simulink model "AFC1_FFNN_trainrp_15_15_15_15_ep_1000_Nor_20250519"  (R2021a)
settings: Solver=ode15s  StartTime=0.0  StopTime=T  MaxStep=.01  RelTol=1e-3
undefined symbols (not defined in the file or in its folder): AF_sensor_tol, fault_time, fuel_inj_tol, kappa_tol, MAF_sensor_tol, pump_tol, tau_ww_tol, x_gain, x_offset, y_gain, y_offset
libraries: neural x66
(part 1 of 3)
Description:
  | Modeling Engine Timing Using Triggered Subsystems
  | 
  | This example presents a model of a four-cylinder spark ignition engine
  | and demonstrates Simulink(R) capabilities to model an internal combustion
  | engine from the throttle to the crankshaft output. We used well-defined
  | physical principles supplemented, where appropriate, with empirical
  | relationships that describe the systems dynamic behavior without
  | introducing unnecessary complexity.
settings Model: ExtModeTrigMode=oneshot  ExtModeArmWhenConnect=off  ExtModeAutoUpdateStatusClock=off  Creator=The MathWorks Inc.  LastModifiedBy=deyun
settings SolverCC: ZeroCrossControl=DisableAll  AlgebraicLoopSolver=TrustRegion
settings DataIOCC: ExternalInput=[t__, u__]  LoadExternalInput=on  SaveFormat=StructureWithTime  SignalLogging=off  DSMLogging=off  ReturnWorkspaceOutputs=off
settings OptimizationCC: BlockReduction=off  BooleanDataType=off  LifeSpan=inf
settings DebuggingCC: SaveWithParameterizedLinksMsg=none  UnderspecifiedInitializationDetection=Classic  MergeDetectMultiDrivingBlocksExec=none  SignalResolutionControl=TryResolveAllWithWarning  ParameterPrecisionLossMsg=none  SFUnexpectedBacktrackingDiag=warning  SFNoUnconditionalDefaultTransitionDiag=warning  SFExecutionAtInitializationDiag=none  ArithmeticOperatorsInVariantConditions=warning
settings HardwareCC: ProdBitPerPointer=32  ProdBitPerSizeT=32  ProdBitPerPtrDiffT=32  ProdLargestAtomicFloat=None  ProdIntDivRoundTo=Undefined  ProdEndianess=Unspecified  ProdWordSize=32  ProdHWDeviceType=32-bit Generic  TargetBitPerLong=64  TargetBitPerPointer=64  TargetBitPerSizeT=64  TargetBitPerPtrDiffT=64  TargetLongLongMode=on  TargetIntDivRoundTo=Zero  TargetEndianess=LittleEndian  TargetWordSize=64  TargetHWDeviceType=MATLAB Host  ProdEqTarget=off
settings ModelReferenceCC: PropagateSignalLabelsOutOfModel=off
settings SFSimCC: SimUseLocalCustomCode=off  CustomCodeUndefinedFunction=UseInterfaceOnly
settings RTWCC: RTWUseLocalCustomCode=off
settings CodeAppCC: StateflowObjectComments=on
settings GRTTargetCC: TargetLangStandard=C89/C90 (ANSI)
settings ConfigComp: CovMetricSettings=d  CovSaveCumulativeToWorkspaceVar=on  CovSaveSingleToWorkspaceVar=on  CovExternalEMLEnable=off

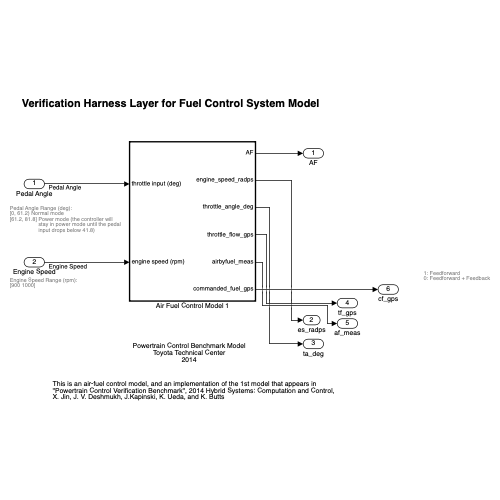
[thumbnail: Simulink's stored preview of the top-level diagram]
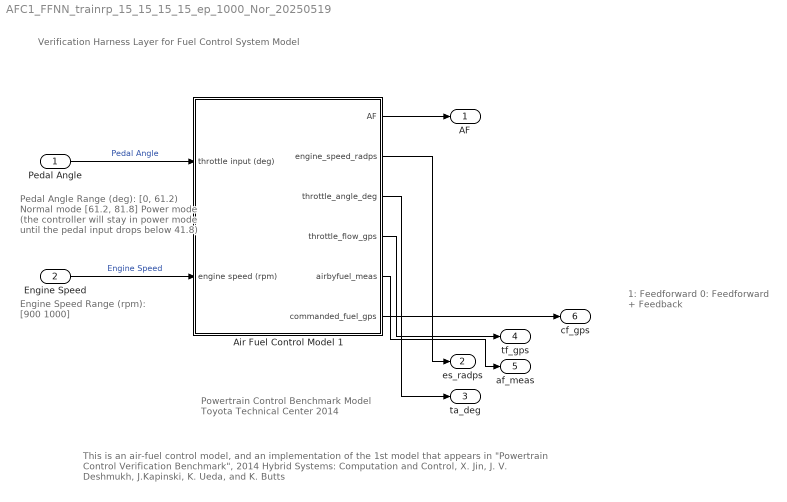
== system AFC1_FFNN_trainrp_15_15_15_15_ep_1000_Nor_20250519 ==
  note: 1: Feedforward
      | 0: Feedforward + Feedback
  note: Pedal Angle Range (deg):
      | [0, 61.2) Normal mode
      | [61.2, 81.8] Power mode (the controller will
      |                    stay in power mode until the pedal
      |                    input drops below 41.8)
  note: This is an air-fuel control model, and an implementation of the 1st model that appears in
      | "Powertrain Control Verification Benchmark", 2014 Hybrid Systems: Computation and Control,
      | X. Jin, J. V. Deshmukh, J.Kapinski, K. Ueda, and K. Butts
  note: Engine Speed Range (rpm):
      | [900 1000]
  note: Powertrain Control Benchmark Model
      | Toyota Technical Center
      | 2014
  note: Verification Harness Layer for Fuel Control System Model
  Pedal Angle : Inport  Interpolate=off
  Engine Speed : Inport  Port=2  Interpolate=off
  Air Fuel Control Model 1 : Subsystem  Priority=1  TreatAsAtomicUnit=on
  AF : Outport  VectorParamsAs1DForOutWhenUnconnected=off
  es_radps : Outport  Port=2
  ta_deg : Outport  Port=3
  tf_gps : Outport  Port=4
  af_meas : Outport  Port=5
  cf_gps : Outport  Port=6
  wires:
  Air Fuel Control Model 1/1(AF) -> AF/1
  Pedal Angle/1 -> Air Fuel Control Model 1/1(throttle input (deg))  "Pedal Angle"
  Engine Speed/1 -> Air Fuel Control Model 1/2(engine speed (rpm))  "Engine Speed"
  Air Fuel Control Model 1/2(engine_speed_radps) -> es_radps/1
  Air Fuel Control Model 1/3(throttle_angle_deg) -> ta_deg/1
  Air Fuel Control Model 1/4(throttle_flow_gps) -> tf_gps/1
  Air Fuel Control Model 1/5(airbyfuel_meas) -> af_meas/1
  Air Fuel Control Model 1/6(commanded_fuel_gps) -> cf_gps/1

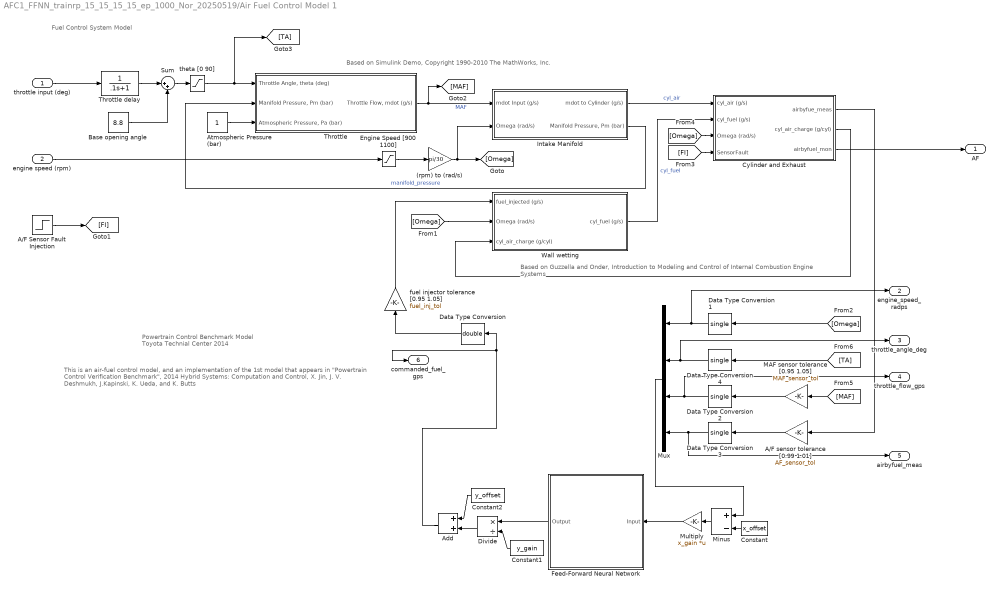
== system AFC1_FFNN_trainrp_15_15_15_15_ep_1000_Nor_20250519/Air Fuel Control Model 1 ==
  note: Based on Simulink Demo, Copyright 1990-2010 The MathWorks, Inc.
  note: Based on Guzzella and Onder, Introduction to Modeling and Control of Internal Combustion Engine Systems
  note: Fuel Control System Model
  note: This is an air-fuel control model, and an implementation of the 1st model that appears in
      | "Powertrain Control Verification Benchmark", 2014 Hybrid Systems: Computation and Control,
      | X. Jin, J. V. Deshmukh, J.Kapinski, K. Ueda, and K. Butts
  note: Powertrain Control Benchmark Model
      | Toyota Technial Center
      | 2014
  throttle input (deg) : Inport  Description=[0, 81.2]
      settings: AttributesFormatString=%<Description>
  engine speed (rpm) : Inport  Description=[900,1100]  Port=2
      settings: AttributesFormatString=%<Description>
  (rpm) to (rad/s) : Gain  Gain=pi/30
  A/F Sensor Fault Injection : Step  Time=fault_time  SampleTime=0
      settings: AttributesFormatString=1: Failure\n0: Normal
  A/F sensor tolerance [0.99 1.01] : Gain  Gain=AF_sensor_tol
  Add : Sum
  Atmospheric Pressure (bar) : Constant
  Base opening angle : Constant  Value=8.8
  Constant : Constant  Value=x_offset
  Constant1 : Constant  Value=y_gain
  Constant2 : Constant  Value=y_offset
  Cylinder and Exhaust : Subsystem
  Data Type Conversion : DataTypeConversion  OutDataTypeStr=double
  Data Type Conversion{1..4} (4 alike) : DataTypeConversion  OutDataTypeStr=single
  Divide : Product  Inputs=*/
  Engine Speed [900 1100] : Saturate  UpperLimit=1100  LowerLimit=900
  Feed-Forward Neural Network : Subsystem
      mask help: Feed-Forward Neural Network
      mask Display: e = 0.06;c1 = [120 150 230]/255;c2 = ([120 150 230]+0)/383;c3 = ([120 150 230]+128)/383;patch([0 1 1 0],[0 0 1 1],c1);patch([0 1 1 1-e 1-e 0+e],[0 0 1 1-e 0+e 0+e],c2);patch([0 0 1 1-e 0+e 0+e],[0 1 1 1-e 1-e 0+e],c3);plot([0 1 1 0 0],[0 0 1 1 0]);fprintf('NNET');port_label('input',1,' Input');port_label('output',1,'Output ');
  Intake Manifold : Subsystem
  MAF sensor tolerance [0.95 1.05] : Gain  Gain=MAF_sensor_tol
  Minus : Sum  Inputs=+-
  Multiply : Gain  Gain=x_gain  Multiplication=Matrix(K*u)
  Mux : Mux
  Sum : Sum  Inputs=|++
  Throttle : Subsystem
  Throttle delay : TransferFcn  Denominator=[.1 1]
  Wall wetting : Subsystem
  fuel injector tolerance [0.95 1.05] : Gain  Gain=fuel_inj_tol
  theta [0 90] : Saturate  UpperLimit=90  LowerLimit=0
  AF : Outport  VectorParamsAs1DForOutWhenUnconnected=off
  engine_speed_radps : Outport  Port=2
  throttle_angle_deg : Outport  Port=3
  throttle_flow_gps : Outport  Port=4
  airbyfuel_meas : Outport  Port=5
  commanded_fuel_gps : Outport  Port=6
  wires:
  (rpm) to (rad/s)/1 -> [Omega], Intake Manifold/2(Omega (rad/s))
  Data Type Conversion/1 -> fuel injector tolerance [0.95 1.05]/1
  theta [0 90]/1 -> Throttle/1("Throttle Angle, theta (deg)"), [TA]
  Engine Speed [900 1100]/1 -> (rpm) to (rad/s)/1
  Cylinder and Exhaust/3("airbyfuel_mon ") -> AF/1
  A/F sensor tolerance [0.99 1.01]/1 -> Data Type Conversion3/1
  [MAF] -> MAF sensor tolerance [0.95 1.05]/1
  Cylinder and Exhaust/1(airbyfue_meas) -> A/F sensor tolerance [0.99 1.01]/1
  Throttle/1("Throttle Flow, mdot (g/s)") -> [MAF], Intake Manifold/1(mdot Input (g/s))  "MAF"
  Intake Manifold/2("Manifold Pressure, Pm (bar)") -> Throttle/2("Manifold Pressure, Pm (bar)")  "manifold_pressure"
  Atmospheric Pressure (bar)/1 -> Throttle/3("Atmospheric Pressure, Pa (bar) ")
  Wall wetting/1(cyl_fuel (g/s)) -> Cylinder and Exhaust/2(cyl_fuel (g/s))  "cyl_fuel"
  Intake Manifold/1(mdot to Cylinder (g/s)) -> Cylinder and Exhaust/1(cyl_air (g/s))  "cyl_air"
  [Omega] -> Cylinder and Exhaust/3(Omega (rad/s))
  [Omega] -> Wall wetting/2(Omega (rad/s))
  Cylinder and Exhaust/2(cyl_air_charge (g/cyl)) -> Wall wetting/3(cyl_air_charge (g/cyl))
  [Omega] -> Data Type Conversion1/1
  fuel injector tolerance [0.95 1.05]/1 -> Wall wetting/1(fuel_injected (g/s))
  MAF sensor tolerance [0.95 1.05]/1 -> Data Type Conversion2/1
  Add/1 -> Data Type Conversion/1, commanded_fuel_gps/1
  A/F Sensor Fault Injection/1 -> [FI]
  [FI] -> Cylinder and Exhaust/4(SensorFault)
  [TA] -> Data Type Conversion4/1
  throttle input (deg)/1 -> Throttle delay/1
  engine speed (rpm)/1 -> Engine Speed [900 1100]/1
  Throttle delay/1 -> Sum/1
  Base opening angle/1 -> Sum/2
  Sum/1 -> theta [0 90]/1
  Data Type Conversion3/1 -> airbyfuel_meas/1, Mux/4
  Data Type Conversion4/1 -> Mux/2, throttle_angle_deg/1
  Data Type Conversion2/1 -> Mux/3, throttle_flow_gps/1
  Data Type Conversion1/1 -> Mux/1, engine_speed_radps/1
  Multiply/1 -> Feed-Forward Neural Network/1(Input)
  Constant/1 -> Minus/2
  Mux/1 -> Minus/1
  Minus/1 -> Multiply/1
  Constant2/1 -> Add/1
  Feed-Forward Neural Network/1(Output) -> Divide/1
  Constant1/1 -> Divide/2
  Divide/1 -> Add/2

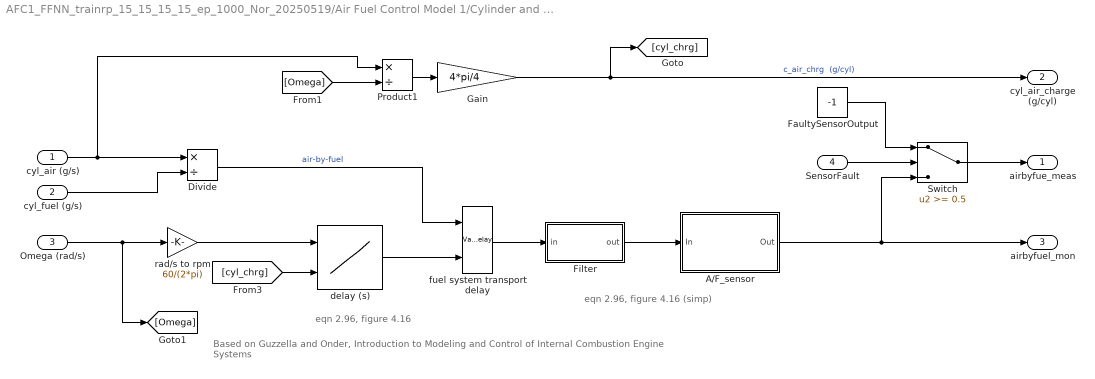
== system AFC1_FFNN_trainrp_15_15_15_15_ep_1000_Nor_20250519/Air Fuel Control Model 1/Cylinder and Exhaust ==
  note: Based on Guzzella and Onder, Introduction to Modeling and Control of Internal Combustion Engine Systems
  note: eqn 2.96, figure 4.16
  note: eqn 2.96, figure 4.16 (simp)
  cyl_air (g/s) : Inport
  cyl_fuel (g/s) : Inport  Port=2
  Omega (rad/s) : Inport  Port=3
  SensorFault : Inport  Port=4
  A/F_sensor : Subsystem
  Divide : Product  Inputs=*/
  FaultySensorOutput : Constant  Value=-1
  Filter : Subsystem
  Gain : Gain  Gain=4*pi/4
  Product1 : Product  Inputs=*/  RndMeth=Zero
  Switch : Switch  Threshold=0.5
  delay (s) : Lookup_n-D  BreakpointsForDimension1=[800,1000,1500,2000,3000]  BreakpointsForDimension2=[0.05,0.15,0.2,0.25]  Table=reshape([0.8,0.6,0.4,0.3,0.2,0.4,0.3,0.2,0.2,0.2,0.3,0.25,0.2,0.2,0.2,0.25,0.2,0.2,0.2,0.2],5,4)  UseLastTableValue=on  RndMeth=Simplest  InputSameDT=on
      settings: InputPortMap=u0,u1
  fuel system transport delay : VariableTransportDelay  VariableDelayType=Variable transport delay  MaximumDelay=10  InitialOutput=14.7  MaximumPoints=20480
  rad/s to rpm : Gain  Gain=60/(2*pi)
  airbyfue_meas : Outport  VectorParamsAs1DForOutWhenUnconnected=off
  cyl_air_charge (g/cyl) : Outport  Port=2  VectorParamsAs1DForOutWhenUnconnected=off
  "airbyfuel_mon " : Outport  Port=3  VectorParamsAs1DForOutWhenUnconnected=off
  wires:
  cyl_air (g/s)/1 -> Divide/1, Product1/1
  [Omega] -> Product1/2
  Product1/1 -> Gain/1
  Gain/1 -> [cyl_chrg], cyl_air_charge (g/cyl)/1  "c_air_chrg  (g/cyl)"
  [cyl_chrg] -> delay (s)/2
  cyl_fuel (g/s)/1 -> Divide/2
  Omega (rad/s)/1 -> [Omega], rad/s to rpm/1
  rad/s to rpm/1 -> delay (s)/1
  delay (s)/1 -> fuel system transport delay/2
  fuel system transport delay/1 -> Filter/1(in)
  Switch/1 -> airbyfue_meas/1
  Divide/1 -> fuel system transport delay/1  "air-by-fuel"
  Filter/1(out) -> A/F_sensor/1(In)
  FaultySensorOutput/1 -> Switch/1
  SensorFault/1 -> Switch/2
  A/F_sensor/1(Out) -> Switch/3, "airbyfuel_mon "/1

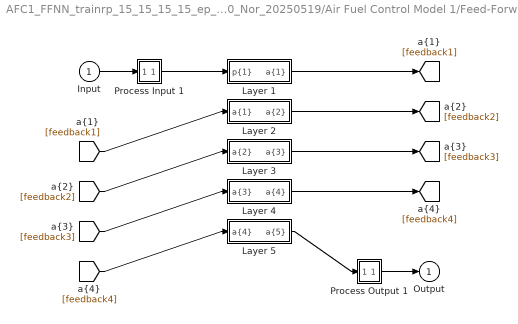
== system AFC1_FFNN_trainrp_15_15_15_15_ep_1000_Nor_20250519/Air Fuel Control Model 1/Feed-Forward Neural Network ==
  Input : Inport  PortDimensions=4
      mask Display: e = 0.06;c1 = [120 230 180]/255;c2 = ([120 230 180]+0)/(256+128);c3 = ([120 230 180]+128)/(256+128);patch([0 1 1 0],[0 0 1 1],c1);patch([0 1 1 1-e 1-e 0+e],[0 0 1 1-e 0+e 0+e],c2);patch([0 0 1 1-e 0+e 0+e],[0 1 1 1-e 1-e 0+e],c3);plot([0 1 1 0 0],[0 0 1 1 0]);
  Layer 1 : Subsystem
      mask Display: e = 0.06;c1 = [120 150 230]/255;c2 = ([120 150 230]+0)/383;c3 = ([120 150 230]+128)/383;patch([0 1 1 0],[0 0 1 1],c1);patch([0 1 1 1-e 1-e 0+e],[0 0 1 1-e 0+e 0+e],c2);patch([0 0 1 1-e 0+e 0+e],[0 1 1 1-e 1-e 0+e],c3);plot([0 1 1 0 0],[0 0 1 1 0]);
  Layer 2 : Subsystem
      mask Display: e = 0.06;c1 = [120 150 230]/255;c2 = ([120 150 230]+0)/383;c3 = ([120 150 230]+128)/383;patch([0 1 1 0],[0 0 1 1],c1);patch([0 1 1 1-e 1-e 0+e],[0 0 1 1-e 0+e 0+e],c2);patch([0 0 1 1-e 0+e 0+e],[0 1 1 1-e 1-e 0+e],c3);plot([0 1 1 0 0],[0 0 1 1 0]);
  Layer 3 : Subsystem
      mask Display: e = 0.06;c1 = [120 150 230]/255;c2 = ([120 150 230]+0)/383;c3 = ([120 150 230]+128)/383;patch([0 1 1 0],[0 0 1 1],c1);patch([0 1 1 1-e 1-e 0+e],[0 0 1 1-e 0+e 0+e],c2);patch([0 0 1 1-e 0+e 0+e],[0 1 1 1-e 1-e 0+e],c3);plot([0 1 1 0 0],[0 0 1 1 0]);
  Layer 4 : Subsystem
      mask Display: e = 0.06;c1 = [120 150 230]/255;c2 = ([120 150 230]+0)/383;c3 = ([120 150 230]+128)/383;patch([0 1 1 0],[0 0 1 1],c1);patch([0 1 1 1-e 1-e 0+e],[0 0 1 1-e 0+e 0+e],c2);patch([0 0 1 1-e 0+e 0+e],[0 1 1 1-e 1-e 0+e],c3);plot([0 1 1 0 0],[0 0 1 1 0]);
  Layer 5 : Subsystem
      mask Display: e = 0.06;c1 = [120 150 230]/255;c2 = ([120 150 230]+0)/383;c3 = ([120 150 230]+128)/383;patch([0 1 1 0],[0 0 1 1],c1);patch([0 1 1 1-e 1-e 0+e],[0 0 1 1-e 0+e 0+e],c2);patch([0 0 1 1-e 0+e 0+e],[0 1 1 1-e 1-e 0+e],c3);plot([0 1 1 0 0],[0 0 1 1 0]);
  Process Input 1 : Subsystem
      mask Display: e = 0.06;c1 = [120 150 230]/255;c2 = ([120 150 230]+0)/383;c3 = ([120 150 230]+128)/383;patch([0 1 1 0],[0 0 1 1],c1);patch([0 1 1 1-e 1-e 0+e],[0 0 1 1-e 0+e 0+e],c2);patch([0 0 1 1-e 0+e 0+e],[0 1 1 1-e 1-e 0+e],c3);plot([0 1 1 0 0],[0 0 1 1 0]);
  Process Output 1 : Subsystem
      mask Display: e = 0.06;c1 = [120 150 230]/255;c2 = ([120 150 230]+0)/383;c3 = ([120 150 230]+128)/383;patch([0 1 1 0],[0 0 1 1],c1);patch([0 1 1 1-e 1-e 0+e],[0 0 1 1-e 0+e 0+e],c2);patch([0 0 1 1-e 0+e 0+e],[0 1 1 1-e 1-e 0+e],c3);plot([0 1 1 0 0],[0 0 1 1 0]);
  Output : Outport  InitialOutput=0
      mask Display: e = 0.06;c1 = [120 230 180]/255;c2 = ([120 230 180]+0)/(256+128);c3 = ([120 230 180]+128)/(256+128);patch([0 1 1 0],[0 0 1 1],c1);patch([0 1 1 1-e 1-e 0+e],[0 0 1 1-e 0+e 0+e],c2);patch([0 0 1 1-e 0+e 0+e],[0 1 1 1-e 1-e 0+e],c3);plot([0 1 1 0 0],[0 0 1 1 0]);
  wires:
  Layer 5/1("a{5}") -> Process Output 1/1(a)
  [feedback4] -> Layer 5/1("a{4} ")
  Layer 4/1("a{4}") -> [feedback4]
  [feedback3] -> Layer 4/1("a{3} ")
  Layer 3/1("a{3}") -> [feedback3]
  [feedback2] -> Layer 3/1("a{2} ")
  Layer 2/1("a{2}") -> [feedback2]
  [feedback1] -> Layer 2/1("a{1} ")
  Layer 1/1("a{1}") -> [feedback1]
  Process Input 1/1(p) -> Layer 1/1("p{1}")
  Process Output 1/1(y) -> Output/1
  Input/1 -> Process Input 1/1(x)

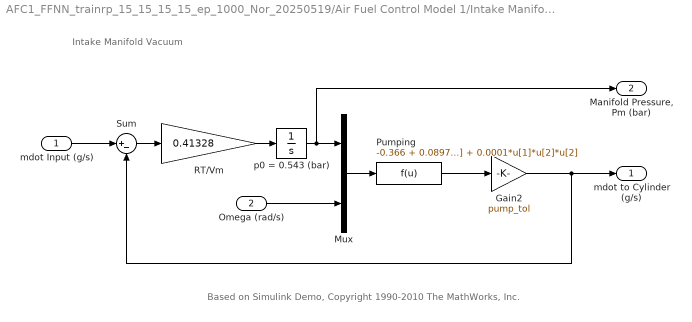
== system AFC1_FFNN_trainrp_15_15_15_15_ep_1000_Nor_20250519/Air Fuel Control Model 1/Intake Manifold ==
  note: Intake Manifold Vacuum
  note: Based on Simulink Demo, Copyright 1990-2010 The MathWorks, Inc.
  mdot Input (g/s) : Inport
  Omega (rad/s) : Inport  Port=2
  Gain2 : Gain  Gain=pump_tol  ParamDataTypeStr=single  OutDataTypeStr=Inherit: Inherit via back propagation  RndMeth=Simplest  SaturateOnIntegerOverflow=on
      settings: AttributesFormatString=pumping tolerance [0.9 1.1]
  Mux : Mux  Inputs=2
  Pumping : Fcn  Expr=-0.366 + 0.08979*u[1]*u[2] - 0.0337*u[2]*u[1]*u[1] + 0.0001*u[1]*u[2]*u[2]
  RT/Vm : Gain  Gain=0.41328  SaturateOnIntegerOverflow=on  OutDataTypeStr=Inherit: Same as input  ParamDataTypeStr=Inherit: Same as input
  Sum : Sum  Inputs=|+-  InputSameDT=on  SaturateOnIntegerOverflow=on  OutDataTypeStr=Inherit: Same as first input
  p0 = 0.543 (bar) : Integrator  InitialCondition=0.982
  mdot to Cylinder (g/s) : Outport  InitialOutput=0  VectorParamsAs1DForOutWhenUnconnected=off
  "Manifold Pressure, Pm (bar)" : Outport  Port=2  InitialOutput=0  VectorParamsAs1DForOutWhenUnconnected=off
  wires:
  mdot Input (g/s)/1 -> Sum/1
  RT/Vm/1 -> p0 = 0.543 (bar)/1
  Omega (rad/s)/1 -> Mux/2
  Mux/1 -> Pumping/1
  p0 = 0.543 (bar)/1 -> Mux/1, "Manifold Pressure, Pm (bar)"/1
  Sum/1 -> RT/Vm/1
  Pumping/1 -> Gain2/1
  Gain2/1 -> Sum/2, mdot to Cylinder (g/s)/1

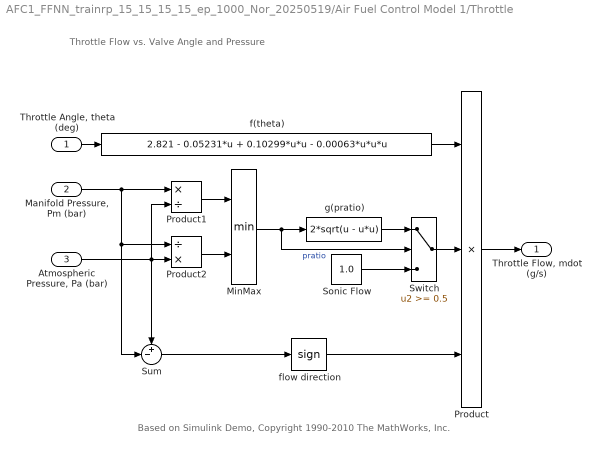
== system AFC1_FFNN_trainrp_15_15_15_15_ep_1000_Nor_20250519/Air Fuel Control Model 1/Throttle ==
  note: Throttle Flow vs. Valve Angle and Pressure
  note: Based on Simulink Demo, Copyright 1990-2010 The MathWorks, Inc.
  "Throttle Angle, theta (deg)" : Inport
  "Manifold Pressure, Pm (bar)" : Inport  Port=2
  "Atmospheric Pressure, Pa (bar) " : Inport  Port=3
  MinMax : MinMax  Inputs=2  InputSameDT=on  SaturateOnIntegerOverflow=on
  Product : Product  Inputs=3  InputSameDT=on  RndMeth=Zero  SaturateOnIntegerOverflow=on  OutDataTypeStr=Inherit: Same as first input
  Product1 : Product  Inputs=*/  InputSameDT=on  RndMeth=Zero  SaturateOnIntegerOverflow=on  OutDataTypeStr=Inherit: Same as first input
  Product2 : Product  Inputs=/*  InputSameDT=on  RndMeth=Zero  SaturateOnIntegerOverflow=on  OutDataTypeStr=Inherit: Same as first input
  "Sonic Flow " : Constant  Value=1.0
  Sum : Sum  Inputs=+-|  InputSameDT=on  SaturateOnIntegerOverflow=on  OutDataTypeStr=Inherit: Same as first input
  Switch : Switch  Threshold=0.5  SaturateOnIntegerOverflow=on  InputSameDT=on
  f(theta) : Fcn  Expr=2.821 - 0.05231*u + 0.10299*u*u - 0.00063*u*u*u
  flow direction : Signum
  g(pratio) : Fcn  Expr=2*sqrt(u - u*u)
  "Throttle Flow, mdot (g/s)" : Outport  InitialOutput=0  VectorParamsAs1DForOutWhenUnconnected=off
  wires:
  "Manifold Pressure, Pm (bar)"/1 -> Sum/2, Product2/1, Product1/1
  Product2/1 -> MinMax/2
  Product1/1 -> MinMax/1
  "Atmospheric Pressure, Pa (bar) "/1 -> Sum/1, Product2/2, Product1/2
  g(pratio)/1 -> Switch/1
  "Sonic Flow "/1 -> Switch/3
  Switch/1 -> Product/2
  flow direction/1 -> Product/3
  Sum/1 -> flow direction/1
  MinMax/1 -> g(pratio)/1, Switch/2  "pratio"
  "Throttle Angle, theta (deg)"/1 -> f(theta)/1
  Product/1 -> "Throttle Flow, mdot (g/s)"/1
  f(theta)/1 -> Product/1

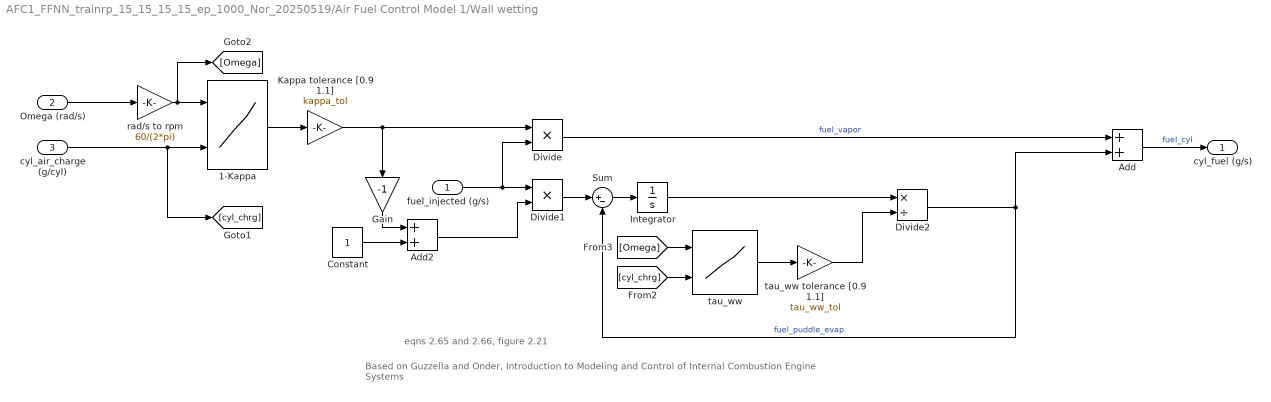
== system AFC1_FFNN_trainrp_15_15_15_15_ep_1000_Nor_20250519/Air Fuel Control Model 1/Wall wetting ==
  note: Based on Guzzella and Onder, Introduction to Modeling and Control of Internal Combustion Engine Systems
  note: eqns 2.65 and 2.66, figure 2.21
  fuel_injected (g/s) : Inport
  Omega (rad/s) : Inport  Port=2
  cyl_air_charge (g/cyl) : Inport  Port=3
  1-Kappa : Lookup_n-D  BreakpointsForDimension1=[1000,1500,2000,2500,3000]  BreakpointsForDimension2=[.1,.2,.3,.4]  Table=reshape([0.8,.7,.7,.8,.9,.7,.66,.65,.73,.85,.66,.66,.63,.66,.8,.6,.6,.6,.6,.7],5,4)  UseLastTableValue=on  RndMeth=Simplest  InputSameDT=on
      settings: InputPortMap=u0,u1
  Add : Sum
  Add2 : Sum
  Constant : Constant
  Divide : Product  Inputs=**
  Divide1 : Product  Inputs=**
  Divide2 : Product  Inputs=*/
  Gain : Gain  Gain=-1
  Integrator : Integrator  InitialCondition=.0112
  Kappa tolerance [0.9 1.1] : Gain  Gain=kappa_tol
  Sum : Sum  Inputs=|+-
  rad/s to rpm : Gain  Gain=60/(2*pi)
  tau_ww : Lookup_n-D  BreakpointsForDimension1=[1000,1500,2000,2500,3000]  BreakpointsForDimension2=[0.1,0.2,0.3,0.4]  Table=reshape([.4,.3,.35,.3,.2,.22,.22,.4,.35,.5,.20,.22,.5,.4,.35,.35,.3,.45,.5,.4],5,4)  UseLastTableValue=on  RndMeth=Simplest  InputSameDT=on
      settings: InputPortMap=u0,u1
  tau_ww tolerance [0.9 1.1] : Gain  Gain=tau_ww_tol
  cyl_fuel (g/s) : Outport  VectorParamsAs1DForOutWhenUnconnected=off
  wires:
  1-Kappa/1 -> Kappa tolerance [0.9 1.1]/1
  fuel_injected (g/s)/1 -> Divide/2, Divide1/1
  Divide/1 -> Add/1  "fuel_vapor"
  Add/1 -> cyl_fuel (g/s)/1  "fuel_cyl"
  Integrator/1 -> Divide2/1
  Divide1/1 -> Sum/1
  Sum/1 -> Integrator/1
  Divide2/1 -> Add/2, Sum/2  "fuel_puddle_evap"
  Add2/1 -> Divide1/2
  cyl_air_charge (g/cyl)/1 -> 1-Kappa/2, [cyl_chrg]
  [cyl_chrg] -> tau_ww/2
  tau_ww/1 -> tau_ww tolerance [0.9 1.1]/1
  Gain/1 -> Add2/1
  Constant/1 -> Add2/2
  rad/s to rpm/1 -> [Omega], 1-Kappa/1
  Omega (rad/s)/1 -> rad/s to rpm/1
  Kappa tolerance [0.9 1.1]/1 -> Divide/1, Gain/1
  tau_ww tolerance [0.9 1.1]/1 -> Divide2/2
  [Omega] -> tau_ww/1

== system AFC1_FFNN_trainrp_15_15_15_15_ep_1000_Nor_20250519/Air Fuel Control Model 1/Cylinder and Exhaust/A//F_sensor ==
  In : Inport
  A/F_sensor : Gain  OutDataTypeStr=double
  Filter : Subsystem
  Out : Outport  VectorParamsAs1DForOutWhenUnconnected=off
  wires:
  A/F_sensor/1 -> Out/1
  In/1 -> Filter/1(In)
  Filter/1(Out) -> A/F_sensor/1

== system AFC1_FFNN_trainrp_15_15_15_15_ep_1000_Nor_20250519/Air Fuel Control Model 1/Cylinder and Exhaust/Filter ==
  in : Inport
  Gain1 : Gain  Gain=10
  Integrator : Integrator  InitialCondition=14.7
  Sum : Sum  Inputs=|+-
  out : Outport  VectorParamsAs1DForOutWhenUnconnected=off
  wires:
  Integrator/1 -> out/1, Sum/2
  in/1 -> Sum/1
  Gain1/1 -> Integrator/1
  Sum/1 -> Gain1/1

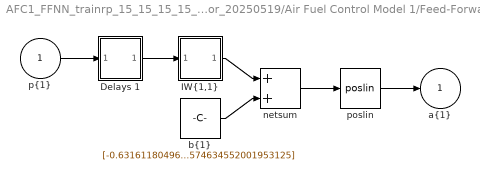
== system AFC1_FFNN_trainrp_15_15_15_15_ep_1000_Nor_20250519/Air Fuel Control Model 1/Feed-Forward Neural Network/Layer 1 ==
  "p{1}" : Inport  PortDimensions=4
      mask Display: e = 0.06;c1 = [120 230 180]/255;c2 = ([120 230 180]+0)/(256+128);c3 = ([120 230 180]+128)/(256+128);patch([0 1 1 0],[0 0 1 1],c1);patch([0 1 1 1-e 1-e 0+e],[0 0 1 1-e 0+e 0+e],c2);patch([0 0 1 1-e 0+e 0+e],[0 1 1 1-e 1-e 0+e],c3);plot([0 1 1 0 0],[0 0 1 1 0]);
  Delays 1 : Subsystem
      mask Display: e = 0.06;c1 = [120 150 230]/255;c2 = ([120 150 230]+0)/383;c3 = ([120 150 230]+128)/383;patch([0 1 1 0],[0 0 1 1],c1);patch([0 1 1 1-e 1-e 0+e],[0 0 1 1-e 0+e 0+e],c2);patch([0 0 1 1-e 0+e 0+e],[0 1 1 1-e 1-e 0+e],c3);plot([0 1 1 0 0],[0 0 1 1 0]);disp('0');
  "IW{1,1}" : Subsystem
      mask Display: e = 0.06;c1 = [120 150 230]/255;c2 = ([120 150 230]+0)/383;c3 = ([120 150 230]+128)/383;patch([0 1 1 0],[0 0 1 1],c1);patch([0 1 1 1-e 1-e 0+e],[0 0 1 1-e 0+e 0+e],c2);patch([0 0 1 1-e 0+e 0+e],[0 1 1 1-e 1-e 0+e],c3);plot([0 1 1 0 0],[0 0 1 1 0]);disp('W');
  "b{1}" : Constant  Value=[-0.63161180496894697711240951321087777614593505859375;0.00962270067570976384008218929011491127312183380126953125;0.0288589178976273209864533697555089020170271396636962890625;-1.0375141343426352857903793847071938216686248779296875;-0.574796933282314181923311480204574763774871826171875;0.8219719903942734884338960910099558532238006591796875;-0.8570943744259109653427231023670174181461334228515625;-0.6103597091916854733284480971633456647396087646484375;-0.734413455287417082928413947229273617267608642578125;-0.274911096506054108967731508528231643140316009521484375;-0.9056216424336513970416717711486853659152984619140625;0.8763539679095886381077207261114381253719329833984375;-0.69068361726473603834364212161744944751262664794921875;-0.8132589664898139947268873584107495844364166259765625;-0.3852662008241598545765782546368427574634552001953125]
      mask Display: e = 0.06;c1 = [120 150 230]/255;c2 = ([120 150 230]+0)/383;c3 = ([120 150 230]+128)/383;patch([0 1 1 0],[0 0 1 1],c1);patch([0 1 1 1-e 1-e 0+e],[0 0 1 1-e 0+e 0+e],c2);patch([0 0 1 1-e 0+e 0+e],[0 1 1 1-e 1-e 0+e],c3);plot([0 1 1 0 0],[0 0 1 1 0]);disp('b');
  netsum : Sum  Inputs=2  InputSameDT=on  SaturateOnIntegerOverflow=on  OutDataTypeStr=Inherit: Same as first input
      mask Display: e = 0.06;c1 = [120 150 230]/255;c2 = ([120 150 230]+0)/383;c3 = ([120 150 230]+128)/383;patch([0 1 1 0],[0 0 1 1],c1);patch([0 1 1 1-e 1-e 0+e],[0 0 1 1-e 0+e 0+e],c2);patch([0 0 1 1-e 0+e 0+e],[0 1 1 1-e 1-e 0+e],c3);plot([0 1 1 0 0],[0 0 1 1 0]);disp('+');
  poslin : neural/Transfer Functions/poslin
  "a{1}" : Outport  InitialOutput=[0;0;0;0;0;0;0;0;0;0;0;0;0;0;0]
      mask Display: e = 0.06;c1 = [120 230 180]/255;c2 = ([120 230 180]+0)/(256+128);c3 = ([120 230 180]+128)/(256+128);patch([0 1 1 0],[0 0 1 1],c1);patch([0 1 1 1-e 1-e 0+e],[0 0 1 1-e 0+e 0+e],c2);patch([0 0 1 1-e 0+e 0+e],[0 1 1 1-e 1-e 0+e],c3);plot([0 1 1 0 0],[0 0 1 1 0]);
  wires:
  poslin/1 -> "a{1}"/1
  netsum/1 -> poslin/1
  "b{1}"/1 -> netsum/2
  "IW{1,1}"/1("iz{1,1}") -> netsum/1
  Delays 1/1("pd{1,1}") -> "IW{1,1}"/1("pd{1,1}")
  "p{1}"/1 -> Delays 1/1("p{1}")

== system AFC1_FFNN_trainrp_15_15_15_15_ep_1000_Nor_20250519/Air Fuel Control Model 1/Feed-Forward Neural Network/Layer 2 ==
  "a{1} " : Inport  PortDimensions=15
      mask Display: e = 0.06;c1 = [120 230 180]/255;c2 = ([120 230 180]+0)/(256+128);c3 = ([120 230 180]+128)/(256+128);patch([0 1 1 0],[0 0 1 1],c1);patch([0 1 1 1-e 1-e 0+e],[0 0 1 1-e 0+e 0+e],c2);patch([0 0 1 1-e 0+e 0+e],[0 1 1 1-e 1-e 0+e],c3);plot([0 1 1 0 0],[0 0 1 1 0]);
  Delays 1 : Subsystem
      mask Display: e = 0.06;c1 = [120 150 230]/255;c2 = ([120 150 230]+0)/383;c3 = ([120 150 230]+128)/383;patch([0 1 1 0],[0 0 1 1],c1);patch([0 1 1 1-e 1-e 0+e],[0 0 1 1-e 0+e 0+e],c2);patch([0 0 1 1-e 0+e 0+e],[0 1 1 1-e 1-e 0+e],c3);plot([0 1 1 0 0],[0 0 1 1 0]);disp('0');
  "LW{2,1}" : Subsystem
      mask Display: e = 0.06;c1 = [120 150 230]/255;c2 = ([120 150 230]+0)/383;c3 = ([120 150 230]+128)/383;patch([0 1 1 0],[0 0 1 1],c1);patch([0 1 1 1-e 1-e 0+e],[0 0 1 1-e 0+e 0+e],c2);patch([0 0 1 1-e 0+e 0+e],[0 1 1 1-e 1-e 0+e],c3);plot([0 1 1 0 0],[0 0 1 1 0]);disp('W');
  "b{2}" : Constant  Value=[0.9642925609619645843650914684985764324665069580078125;0.67125541175712211128256967640481889247894287109375;0.10408553167570726294410832224457408301532268524169921875;-0.189928808479492727823156883459887467324733734130859375;-0.377128510325493826460530044641927815973758697509765625;0.1485391877348999634111947898418293334543704986572265625;-0.5426610357889971592015854184865020215511322021484375;-0.6003893385198704191196839019539766013622283935546875;0.83673894348263300191348434964311309158802032470703125;0.84107240300872609939375479370937682688236236572265625;0.360425029571680266560207428483408875763416290283203125;-0.02163834313229549832779952112105092965066432952880859375;-0.10199940059879332443504296179526136256754398345947265625;-0.288475835591650964229160081231384538114070892333984375;0.77261343131387361093942445222637616097927093505859375]
      mask Display: e = 0.06;c1 = [120 150 230]/255;c2 = ([120 150 230]+0)/383;c3 = ([120 150 230]+128)/383;patch([0 1 1 0],[0 0 1 1],c1);patch([0 1 1 1-e 1-e 0+e],[0 0 1 1-e 0+e 0+e],c2);patch([0 0 1 1-e 0+e 0+e],[0 1 1 1-e 1-e 0+e],c3);plot([0 1 1 0 0],[0 0 1 1 0]);disp('b');
  netsum : Sum  Inputs=2  InputSameDT=on  SaturateOnIntegerOverflow=on  OutDataTypeStr=Inherit: Same as first input
      mask Display: e = 0.06;c1 = [120 150 230]/255;c2 = ([120 150 230]+0)/383;c3 = ([120 150 230]+128)/383;patch([0 1 1 0],[0 0 1 1],c1);patch([0 1 1 1-e 1-e 0+e],[0 0 1 1-e 0+e 0+e],c2);patch([0 0 1 1-e 0+e 0+e],[0 1 1 1-e 1-e 0+e],c3);plot([0 1 1 0 0],[0 0 1 1 0]);disp('+');
  poslin : neural/Transfer Functions/poslin
  "a{2}" : Outport  InitialOutput=[0;0;0;0;0;0;0;0;0;0;0;0;0;0;0]
      mask Display: e = 0.06;c1 = [120 230 180]/255;c2 = ([120 230 180]+0)/(256+128);c3 = ([120 230 180]+128)/(256+128);patch([0 1 1 0],[0 0 1 1],c1);patch([0 1 1 1-e 1-e 0+e],[0 0 1 1-e 0+e 0+e],c2);patch([0 0 1 1-e 0+e 0+e],[0 1 1 1-e 1-e 0+e],c3);plot([0 1 1 0 0],[0 0 1 1 0]);
  wires:
  poslin/1 -> "a{2}"/1
  netsum/1 -> poslin/1
  "b{2}"/1 -> netsum/2
  "LW{2,1}"/1("lz{2,1}") -> netsum/1
  Delays 1/1("pd{2,1}") -> "LW{2,1}"/1("ad{2,1}")
  "a{1} "/1 -> Delays 1/1("p{2}")

== system AFC1_FFNN_trainrp_15_15_15_15_ep_1000_Nor_20250519/Air Fuel Control Model 1/Feed-Forward Neural Network/Layer 3 ==
  "a{2} " : Inport  PortDimensions=15
      mask Display: e = 0.06;c1 = [120 230 180]/255;c2 = ([120 230 180]+0)/(256+128);c3 = ([120 230 180]+128)/(256+128);patch([0 1 1 0],[0 0 1 1],c1);patch([0 1 1 1-e 1-e 0+e],[0 0 1 1-e 0+e 0+e],c2);patch([0 0 1 1-e 0+e 0+e],[0 1 1 1-e 1-e 0+e],c3);plot([0 1 1 0 0],[0 0 1 1 0]);
  Delays 1 : Subsystem
      mask Display: e = 0.06;c1 = [120 150 230]/255;c2 = ([120 150 230]+0)/383;c3 = ([120 150 230]+128)/383;patch([0 1 1 0],[0 0 1 1],c1);patch([0 1 1 1-e 1-e 0+e],[0 0 1 1-e 0+e 0+e],c2);patch([0 0 1 1-e 0+e 0+e],[0 1 1 1-e 1-e 0+e],c3);plot([0 1 1 0 0],[0 0 1 1 0]);disp('0');
  "LW{3,2}" : Subsystem
      mask Display: e = 0.06;c1 = [120 150 230]/255;c2 = ([120 150 230]+0)/383;c3 = ([120 150 230]+128)/383;patch([0 1 1 0],[0 0 1 1],c1);patch([0 1 1 1-e 1-e 0+e],[0 0 1 1-e 0+e 0+e],c2);patch([0 0 1 1-e 0+e 0+e],[0 1 1 1-e 1-e 0+e],c3);plot([0 1 1 0 0],[0 0 1 1 0]);disp('W');
  "b{3}" : Constant  Value=[-0.8795452320810144275498032584437169134616851806640625;-0.7692529834342003436375989622320048511028289794921875;0.73051597519094191302002627708134241402149200439453125;0.41907789382992965965257781135733239352703094482421875;-0.7662077060546554907460858885315246880054473876953125;-0.2196623107028083665692719250728259794414043426513671875;-1.060990963495740846411763413925655186176300048828125;-0.64792235720543367438750692599569447338581085205078125;-0.9352196597747906015030139315058477222919464111328125;-0.254729877874980192853371363526093773543834686279296875;-0.74529099887340632957233310662559233605861663818359375;-0.303984680567773057902059008483774960041046142578125;-1.011483091384547616797817681799642741680145263671875;0.7081472302143889674397314593079499900341033935546875;-0.727379727718625357368864570162259042263031005859375]
      mask Display: e = 0.06;c1 = [120 150 230]/255;c2 = ([120 150 230]+0)/383;c3 = ([120 150 230]+128)/383;patch([0 1 1 0],[0 0 1 1],c1);patch([0 1 1 1-e 1-e 0+e],[0 0 1 1-e 0+e 0+e],c2);patch([0 0 1 1-e 0+e 0+e],[0 1 1 1-e 1-e 0+e],c3);plot([0 1 1 0 0],[0 0 1 1 0]);disp('b');
  netsum : Sum  Inputs=2  InputSameDT=on  SaturateOnIntegerOverflow=on  OutDataTypeStr=Inherit: Same as first input
      mask Display: e = 0.06;c1 = [120 150 230]/255;c2 = ([120 150 230]+0)/383;c3 = ([120 150 230]+128)/383;patch([0 1 1 0],[0 0 1 1],c1);patch([0 1 1 1-e 1-e 0+e],[0 0 1 1-e 0+e 0+e],c2);patch([0 0 1 1-e 0+e 0+e],[0 1 1 1-e 1-e 0+e],c3);plot([0 1 1 0 0],[0 0 1 1 0]);disp('+');
  poslin : neural/Transfer Functions/poslin
  "a{3}" : Outport  InitialOutput=[0;0;0;0;0;0;0;0;0;0;0;0;0;0;0]
      mask Display: e = 0.06;c1 = [120 230 180]/255;c2 = ([120 230 180]+0)/(256+128);c3 = ([120 230 180]+128)/(256+128);patch([0 1 1 0],[0 0 1 1],c1);patch([0 1 1 1-e 1-e 0+e],[0 0 1 1-e 0+e 0+e],c2);patch([0 0 1 1-e 0+e 0+e],[0 1 1 1-e 1-e 0+e],c3);plot([0 1 1 0 0],[0 0 1 1 0]);
  wires:
  poslin/1 -> "a{3}"/1
  netsum/1 -> poslin/1
  "b{3}"/1 -> netsum/2
  "LW{3,2}"/1("lz{3,2}") -> netsum/1
  Delays 1/1("pd{3,2}") -> "LW{3,2}"/1("ad{3,2}")
  "a{2} "/1 -> Delays 1/1("p{3}")

== system AFC1_FFNN_trainrp_15_15_15_15_ep_1000_Nor_20250519/Air Fuel Control Model 1/Feed-Forward Neural Network/Layer 4 ==
  "a{3} " : Inport  PortDimensions=15
      mask Display: e = 0.06;c1 = [120 230 180]/255;c2 = ([120 230 180]+0)/(256+128);c3 = ([120 230 180]+128)/(256+128);patch([0 1 1 0],[0 0 1 1],c1);patch([0 1 1 1-e 1-e 0+e],[0 0 1 1-e 0+e 0+e],c2);patch([0 0 1 1-e 0+e 0+e],[0 1 1 1-e 1-e 0+e],c3);plot([0 1 1 0 0],[0 0 1 1 0]);
  Delays 1 : Subsystem
      mask Display: e = 0.06;c1 = [120 150 230]/255;c2 = ([120 150 230]+0)/383;c3 = ([120 150 230]+128)/383;patch([0 1 1 0],[0 0 1 1],c1);patch([0 1 1 1-e 1-e 0+e],[0 0 1 1-e 0+e 0+e],c2);patch([0 0 1 1-e 0+e 0+e],[0 1 1 1-e 1-e 0+e],c3);plot([0 1 1 0 0],[0 0 1 1 0]);disp('0');
  "LW{4,3}" : Subsystem
      mask Display: e = 0.06;c1 = [120 150 230]/255;c2 = ([120 150 230]+0)/383;c3 = ([120 150 230]+128)/383;patch([0 1 1 0],[0 0 1 1],c1);patch([0 1 1 1-e 1-e 0+e],[0 0 1 1-e 0+e 0+e],c2);patch([0 0 1 1-e 0+e 0+e],[0 1 1 1-e 1-e 0+e],c3);plot([0 1 1 0 0],[0 0 1 1 0]);disp('W');
  "b{4}" : Constant  Value=[0.6430190038915777339667556589120067656040191650390625;-0.88860416367711370089210731748607940971851348876953125;0.8016549747879573306619249706272967159748077392578125;-0.74196661172648215032410234925919212400913238525390625;-0.09539261572522128584949996366049163043498992919921875;-0.681714695614326959827167229377664625644683837890625;0.203616360248826067103067316566011868417263031005859375;-0.990840752105353050893654653918929398059844970703125;0.4496629313994926491204751073382794857025146484375;0.60501845291656464187468600357533432543277740478515625;0.775199883043331539056453038938343524932861328125;0.9928375063025234315006173346773721277713775634765625;0.07793445071594727602271035493686213158071041107177734375;-0.54085781593318127402625350441667251288890838623046875;-1.3945629761575286664765371824614703655242919921875]
      mask Display: e = 0.06;c1 = [120 150 230]/255;c2 = ([120 150 230]+0)/383;c3 = ([120 150 230]+128)/383;patch([0 1 1 0],[0 0 1 1],c1);patch([0 1 1 1-e 1-e 0+e],[0 0 1 1-e 0+e 0+e],c2);patch([0 0 1 1-e 0+e 0+e],[0 1 1 1-e 1-e 0+e],c3);plot([0 1 1 0 0],[0 0 1 1 0]);disp('b');
  netsum : Sum  Inputs=2  InputSameDT=on  SaturateOnIntegerOverflow=on  OutDataTypeStr=Inherit: Same as first input
      mask Display: e = 0.06;c1 = [120 150 230]/255;c2 = ([120 150 230]+0)/383;c3 = ([120 150 230]+128)/383;patch([0 1 1 0],[0 0 1 1],c1);patch([0 1 1 1-e 1-e 0+e],[0 0 1 1-e 0+e 0+e],c2);patch([0 0 1 1-e 0+e 0+e],[0 1 1 1-e 1-e 0+e],c3);plot([0 1 1 0 0],[0 0 1 1 0]);disp('+');
  poslin : neural/Transfer Functions/poslin
  "a{4}" : Outport  InitialOutput=[0;0;0;0;0;0;0;0;0;0;0;0;0;0;0]
      mask Display: e = 0.06;c1 = [120 230 180]/255;c2 = ([120 230 180]+0)/(256+128);c3 = ([120 230 180]+128)/(256+128);patch([0 1 1 0],[0 0 1 1],c1);patch([0 1 1 1-e 1-e 0+e],[0 0 1 1-e 0+e 0+e],c2);patch([0 0 1 1-e 0+e 0+e],[0 1 1 1-e 1-e 0+e],c3);plot([0 1 1 0 0],[0 0 1 1 0]);
  wires:
  poslin/1 -> "a{4}"/1
  netsum/1 -> poslin/1
  "b{4}"/1 -> netsum/2
  "LW{4,3}"/1("lz{4,3}") -> netsum/1
  Delays 1/1("pd{4,3}") -> "LW{4,3}"/1("ad{4,3}")
  "a{3} "/1 -> Delays 1/1("p{4}")

== system AFC1_FFNN_trainrp_15_15_15_15_ep_1000_Nor_20250519/Air Fuel Control Model 1/Feed-Forward Neural Network/Layer 5 ==
  "a{4} " : Inport  PortDimensions=15
      mask Display: e = 0.06;c1 = [120 230 180]/255;c2 = ([120 230 180]+0)/(256+128);c3 = ([120 230 180]+128)/(256+128);patch([0 1 1 0],[0 0 1 1],c1);patch([0 1 1 1-e 1-e 0+e],[0 0 1 1-e 0+e 0+e],c2);patch([0 0 1 1-e 0+e 0+e],[0 1 1 1-e 1-e 0+e],c3);plot([0 1 1 0 0],[0 0 1 1 0]);
  Delays 1 : Subsystem
      mask Display: e = 0.06;c1 = [120 150 230]/255;c2 = ([120 150 230]+0)/383;c3 = ([120 150 230]+128)/383;patch([0 1 1 0],[0 0 1 1],c1);patch([0 1 1 1-e 1-e 0+e],[0 0 1 1-e 0+e 0+e],c2);patch([0 0 1 1-e 0+e 0+e],[0 1 1 1-e 1-e 0+e],c3);plot([0 1 1 0 0],[0 0 1 1 0]);disp('0');
  "LW{5,4}" : Subsystem
      mask Display: e = 0.06;c1 = [120 150 230]/255;c2 = ([120 150 230]+0)/383;c3 = ([120 150 230]+128)/383;patch([0 1 1 0],[0 0 1 1],c1);patch([0 1 1 1-e 1-e 0+e],[0 0 1 1-e 0+e 0+e],c2);patch([0 0 1 1-e 0+e 0+e],[0 1 1 1-e 1-e 0+e],c3);plot([0 1 1 0 0],[0 0 1 1 0]);disp('W');
  "b{5}" : Constant  Value=0.02407306573906788094152631174438283778727054595947265625
      mask Display: e = 0.06;c1 = [120 150 230]/255;c2 = ([120 150 230]+0)/383;c3 = ([120 150 230]+128)/383;patch([0 1 1 0],[0 0 1 1],c1);patch([0 1 1 1-e 1-e 0+e],[0 0 1 1-e 0+e 0+e],c2);patch([0 0 1 1-e 0+e 0+e],[0 1 1 1-e 1-e 0+e],c3);plot([0 1 1 0 0],[0 0 1 1 0]);disp('b');
  netsum : Sum  Inputs=2  InputSameDT=on  SaturateOnIntegerOverflow=on  OutDataTypeStr=Inherit: Same as first input
      mask Display: e = 0.06;c1 = [120 150 230]/255;c2 = ([120 150 230]+0)/383;c3 = ([120 150 230]+128)/383;patch([0 1 1 0],[0 0 1 1],c1);patch([0 1 1 1-e 1-e 0+e],[0 0 1 1-e 0+e 0+e],c2);patch([0 0 1 1-e 0+e 0+e],[0 1 1 1-e 1-e 0+e],c3);plot([0 1 1 0 0],[0 0 1 1 0]);disp('+');
  purelin : neural/Transfer Functions/purelin
  "a{5}" : Outport  InitialOutput=0
      mask Display: e = 0.06;c1 = [120 230 180]/255;c2 = ([120 230 180]+0)/(256+128);c3 = ([120 230 180]+128)/(256+128);patch([0 1 1 0],[0 0 1 1],c1);patch([0 1 1 1-e 1-e 0+e],[0 0 1 1-e 0+e 0+e],c2);patch([0 0 1 1-e 0+e 0+e],[0 1 1 1-e 1-e 0+e],c3);plot([0 1 1 0 0],[0 0 1 1 0]);
  wires:
  purelin/1 -> "a{5}"/1
  netsum/1 -> purelin/1
  "b{5}"/1 -> netsum/2
  "LW{5,4}"/1("lz{5,4}") -> netsum/1
  Delays 1/1("pd{5,4}") -> "LW{5,4}"/1("ad{5,4}")
  "a{4} "/1 -> Delays 1/1("p{5}")

== system AFC1_FFNN_trainrp_15_15_15_15_ep_1000_Nor_20250519/Air Fuel Control Model 1/Feed-Forward Neural Network/Process Input 1 ==
  x : Inport  PortDimensions=4
      mask Display: e = 0.06;c1 = [120 230 180]/255;c2 = ([120 230 180]+0)/(256+128);c3 = ([120 230 180]+128)/(256+128);patch([0 1 1 0],[0 0 1 1],c1);patch([0 1 1 1-e 1-e 0+e],[0 0 1 1-e 0+e 0+e],c2);patch([0 0 1 1-e 0+e 0+e],[0 1 1 1-e 1-e 0+e],c3);plot([0 1 1 0 0],[0 0 1 1 0]);
  p : Outport  PortDimensions=4
      mask Display: e = 0.06;c1 = [120 230 180]/255;c2 = ([120 230 180]+0)/(256+128);c3 = ([120 230 180]+128)/(256+128);patch([0 1 1 0],[0 0 1 1],c1);patch([0 1 1 1-e 1-e 0+e],[0 0 1 1-e 0+e 0+e],c2);patch([0 0 1 1-e 0+e 0+e],[0 1 1 1-e 1-e 0+e],c3);plot([0 1 1 0 0],[0 0 1 1 0]);
  wires:
  x/1 -> p/1

== system AFC1_FFNN_trainrp_15_15_15_15_ep_1000_Nor_20250519/Air Fuel Control Model 1/Feed-Forward Neural Network/Process Output 1 ==
  a : Inport  PortDimensions=1
      mask Display: e = 0.06;c1 = [120 230 180]/255;c2 = ([120 230 180]+0)/(256+128);c3 = ([120 230 180]+128)/(256+128);patch([0 1 1 0],[0 0 1 1],c1);patch([0 1 1 1-e 1-e 0+e],[0 0 1 1-e 0+e 0+e],c2);patch([0 0 1 1-e 0+e 0+e],[0 1 1 1-e 1-e 0+e],c3);plot([0 1 1 0 0],[0 0 1 1 0]);
  y : Outport  PortDimensions=1
      mask Display: e = 0.06;c1 = [120 230 180]/255;c2 = ([120 230 180]+0)/(256+128);c3 = ([120 230 180]+128)/(256+128);patch([0 1 1 0],[0 0 1 1],c1);patch([0 1 1 1-e 1-e 0+e],[0 0 1 1-e 0+e 0+e],c2);patch([0 0 1 1-e 0+e 0+e],[0 1 1 1-e 1-e 0+e],c3);plot([0 1 1 0 0],[0 0 1 1 0]);
  wires:
  a/1 -> y/1

== system AFC1_FFNN_trainrp_15_15_15_15_ep_1000_Nor_20250519/Air Fuel Control Model 1/Cylinder and Exhaust/A//F_sensor/Filter ==
  In : Inport
  Gain : Gain  Gain=50
  Integrator : Integrator  InitialCondition=14.7
  Sum : Sum  Inputs=|+-
  Out : Outport  VectorParamsAs1DForOutWhenUnconnected=off
  wires:
  Integrator/1 -> Out/1, Sum/2
  In/1 -> Sum/1
  Gain/1 -> Integrator/1
  Sum/1 -> Gain/1

== system AFC1_FFNN_trainrp_15_15_15_15_ep_1000_Nor_20250519/Air Fuel Control Model 1/Feed-Forward Neural Network/Layer 1/Delays 1 ==
  "p{1}" : Inport  PortDimensions=4
      mask Display: e = 0.06;c1 = [120 230 180]/255;c2 = ([120 230 180]+0)/(256+128);c3 = ([120 230 180]+128)/(256+128);patch([0 1 1 0],[0 0 1 1],c1);patch([0 1 1 1-e 1-e 0+e],[0 0 1 1-e 0+e 0+e],c2);patch([0 0 1 1-e 0+e 0+e],[0 1 1 1-e 1-e 0+e],c3);plot([0 1 1 0 0],[0 0 1 1 0]);
  mux : Mux  Inputs=1
      mask Display: e = 0.06;c1 = [120 150 230]/255;c2 = ([120 150 230]+0)/383;c3 = ([120 150 230]+128)/383;patch([0 1 1 0],[0 0 1 1],c1);patch([0 1 1 1-e 1-e 0+e],[0 0 1 1-e 0+e 0+e],c2);patch([0 0 1 1-e 0+e 0+e],[0 1 1 1-e 1-e 0+e],c3);plot([0 1 1 0 0],[0 0 1 1 0]);disp('Mux')
  "pd{1,1}" : Outport
      mask Display: e = 0.06;c1 = [120 230 180]/255;c2 = ([120 230 180]+0)/(256+128);c3 = ([120 230 180]+128)/(256+128);patch([0 1 1 0],[0 0 1 1],c1);patch([0 1 1 1-e 1-e 0+e],[0 0 1 1-e 0+e 0+e],c2);patch([0 0 1 1-e 0+e 0+e],[0 1 1 1-e 1-e 0+e],c3);plot([0 1 1 0 0],[0 0 1 1 0]);
  wires:
  mux/1 -> "pd{1,1}"/1
  "p{1}"/1 -> mux/1

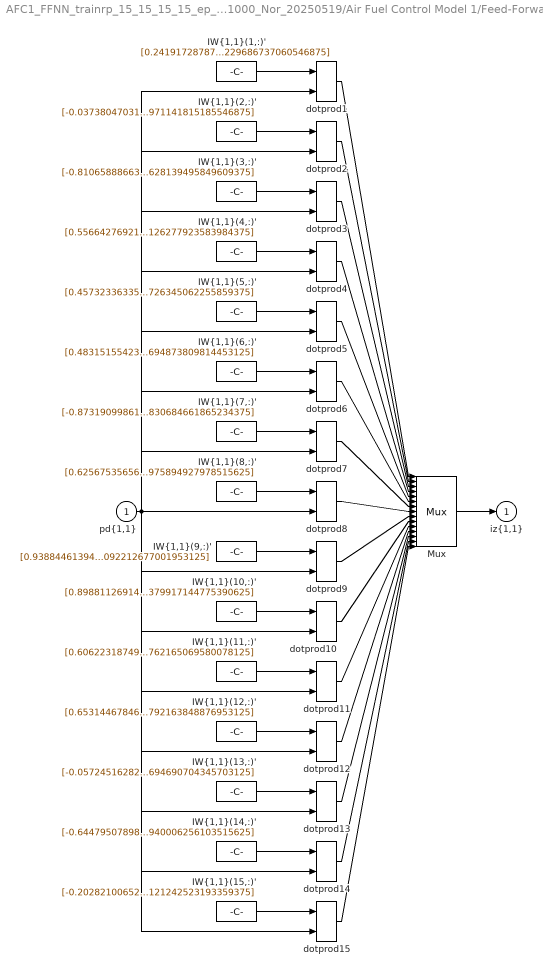
== system AFC1_FFNN_trainrp_15_15_15_15_ep_1000_Nor_20250519/Air Fuel Control Model 1/Feed-Forward Neural Network/Layer 1/IW{1,1} ==
  "pd{1,1}" : Inport  PortDimensions=4
      mask Display: e = 0.06;c1 = [120 230 180]/255;c2 = ([120 230 180]+0)/(256+128);c3 = ([120 230 180]+128)/(256+128);patch([0 1 1 0],[0 0 1 1],c1);patch([0 1 1 1-e 1-e 0+e],[0 0 1 1-e 0+e 0+e],c2);patch([0 0 1 1-e 0+e 0+e],[0 1 1 1-e 1-e 0+e],c3);plot([0 1 1 0 0],[0 0 1 1 0]);
  "IW{1,1}(1,:)'" : Constant  Value=[0.241917287870616615208518851432017982006072998046875;-0.7321374980240575869316899115801788866519927978515625;-0.6457849324217816988635831876308657228946685791015625;-0.643766092226467190329231016221456229686737060546875]
      mask Display: e = 0.06;c1 = [120 150 230]/255;c2 = ([120 150 230]+0)/383;c3 = ([120 150 230]+128)/383;patch([0 1 1 0],[0 0 1 1],c1);patch([0 1 1 1-e 1-e 0+e],[0 0 1 1-e 0+e 0+e],c2);patch([0 0 1 1-e 0+e 0+e],[0 1 1 1-e 1-e 0+e],c3);plot([0 1 1 0 0],[0 0 1 1 0]);disp('Weights');
  "IW{1,1}(10,:)'" : Constant  Value=[0.89881126914582598619318787314114160835742950439453125;0.6283704489907597778852732517407275736331939697265625;-0.55359868381541510462540145454113371670246124267578125;-0.2093283477983797491450701500070863403379917144775390625]
      mask Display: e = 0.06;c1 = [120 150 230]/255;c2 = ([120 150 230]+0)/383;c3 = ([120 150 230]+128)/383;patch([0 1 1 0],[0 0 1 1],c1);patch([0 1 1 1-e 1-e 0+e],[0 0 1 1-e 0+e 0+e],c2);patch([0 0 1 1-e 0+e 0+e],[0 1 1 1-e 1-e 0+e],c3);plot([0 1 1 0 0],[0 0 1 1 0]);disp('Weights');
  "IW{1,1}(11,:)'" : Constant  Value=[0.60622318749349968225459406312438659369945526123046875;0.1920875245654551921603570008301176130771636962890625;-0.0960056259084546559368078533225343562662601470947265625;1.0779332249872617399688579098437912762165069580078125]
      mask Display: e = 0.06;c1 = [120 150 230]/255;c2 = ([120 150 230]+0)/383;c3 = ([120 150 230]+128)/383;patch([0 1 1 0],[0 0 1 1],c1);patch([0 1 1 1-e 1-e 0+e],[0 0 1 1-e 0+e 0+e],c2);patch([0 0 1 1-e 0+e 0+e],[0 1 1 1-e 1-e 0+e],c3);plot([0 1 1 0 0],[0 0 1 1 0]);disp('Weights');
  "IW{1,1}(12,:)'" : Constant  Value=[0.6531446784684005191223832298419438302516937255859375;0.76714139702899941664071548075298778712749481201171875;0.019156088563747793174218969625144382007420063018798828125;-0.368245072466052481008347285751369781792163848876953125]
      mask Display: e = 0.06;c1 = [120 150 230]/255;c2 = ([120 150 230]+0)/383;c3 = ([120 150 230]+128)/383;patch([0 1 1 0],[0 0 1 1],c1);patch([0 1 1 1-e 1-e 0+e],[0 0 1 1-e 0+e 0+e],c2);patch([0 0 1 1-e 0+e 0+e],[0 1 1 1-e 1-e 0+e],c3);plot([0 1 1 0 0],[0 0 1 1 0]);disp('Weights');
  "IW{1,1}(13,:)'" : Constant  Value=[-0.05724516282485019036396778346897917799651622772216796875;-0.388241611345477799499548154926742427051067352294921875;0.443914156983913177345613121360656805336475372314453125;0.407092147403434634345131826194119639694690704345703125]
      mask Display: e = 0.06;c1 = [120 150 230]/255;c2 = ([120 150 230]+0)/383;c3 = ([120 150 230]+128)/383;patch([0 1 1 0],[0 0 1 1],c1);patch([0 1 1 1-e 1-e 0+e],[0 0 1 1-e 0+e 0+e],c2);patch([0 0 1 1-e 0+e 0+e],[0 1 1 1-e 1-e 0+e],c3);plot([0 1 1 0 0],[0 0 1 1 0]);disp('Weights');
  "IW{1,1}(14,:)'" : Constant  Value=[-0.644795078988269931841159632313065230846405029296875;-0.1079467038897943265141066149226389825344085693359375;0.636408077815341588490127833210863173007965087890625;0.4725349111932770629351807656348682940006256103515625]
      mask Display: e = 0.06;c1 = [120 150 230]/255;c2 = ([120 150 230]+0)/383;c3 = ([120 150 230]+128)/383;patch([0 1 1 0],[0 0 1 1],c1);patch([0 1 1 1-e 1-e 0+e],[0 0 1 1-e 0+e 0+e],c2);patch([0 0 1 1-e 0+e 0+e],[0 1 1 1-e 1-e 0+e],c3);plot([0 1 1 0 0],[0 0 1 1 0]);disp('Weights');
  "IW{1,1}(15,:)'" : Constant  Value=[-0.2028210065283138074931912342435680329799652099609375;-0.891521031117740836435814344440586864948272705078125;-0.799556919609016869543438588152639567852020263671875;0.12372285056327481100879595032893121242523193359375]
      mask Display: e = 0.06;c1 = [120 150 230]/255;c2 = ([120 150 230]+0)/383;c3 = ([120 150 230]+128)/383;patch([0 1 1 0],[0 0 1 1],c1);patch([0 1 1 1-e 1-e 0+e],[0 0 1 1-e 0+e 0+e],c2);patch([0 0 1 1-e 0+e 0+e],[0 1 1 1-e 1-e 0+e],c3);plot([0 1 1 0 0],[0 0 1 1 0]);disp('Weights');
  "IW{1,1}(2,:)'" : Constant  Value=[-0.03738047031760365068731033488802495412528514862060546875;-1.1230209025100970077204465269460342824459075927734375;0.140816123921948810338022894939058460295200347900390625;-0.465530173035839378581357550501707009971141815185546875]
      mask Display: e = 0.06;c1 = [120 150 230]/255;c2 = ([120 150 230]+0)/383;c3 = ([120 150 230]+128)/383;patch([0 1 1 0],[0 0 1 1],c1);patch([0 1 1 1-e 1-e 0+e],[0 0 1 1-e 0+e 0+e],c2);patch([0 0 1 1-e 0+e 0+e],[0 1 1 1-e 1-e 0+e],c3);plot([0 1 1 0 0],[0 0 1 1 0]);disp('Weights');
  "IW{1,1}(3,:)'" : Constant  Value=[-0.8106588866396204906550337909720838069915771484375;1.0331541708985179095492412670864723622798919677734375;-0.1447935136725519156275510113118798471987247467041015625;-0.07934547113187927214195127589846379123628139495849609375]
      mask Display: e = 0.06;c1 = [120 150 230]/255;c2 = ([120 150 230]+0)/383;c3 = ([120 150 230]+128)/383;patch([0 1 1 0],[0 0 1 1],c1);patch([0 1 1 1-e 1-e 0+e],[0 0 1 1-e 0+e 0+e],c2);patch([0 0 1 1-e 0+e 0+e],[0 1 1 1-e 1-e 0+e],c3);plot([0 1 1 0 0],[0 0 1 1 0]);disp('Weights');
  "IW{1,1}(4,:)'" : Constant  Value=[0.55664276921649935570002298845793120563030242919921875;-0.703147870827215637490326116676442325115203857421875;0.491212275668599096523081470877514220774173736572265625;-0.261988652677441535843172459863126277923583984375]
      mask Display: e = 0.06;c1 = [120 150 230]/255;c2 = ([120 150 230]+0)/383;c3 = ([120 150 230]+128)/383;patch([0 1 1 0],[0 0 1 1],c1);patch([0 1 1 1-e 1-e 0+e],[0 0 1 1-e 0+e 0+e],c2);patch([0 0 1 1-e 0+e 0+e],[0 1 1 1-e 1-e 0+e],c3);plot([0 1 1 0 0],[0 0 1 1 0]);disp('Weights');
  "IW{1,1}(5,:)'" : Constant  Value=[0.457323363356542333946208600536920130252838134765625;-0.408932331049287167701322687207721173763275146484375;-0.763689603106578740465693044825457036495208740234375;-0.3283020506461509224749306667945347726345062255859375]
      mask Display: e = 0.06;c1 = [120 150 230]/255;c2 = ([120 150 230]+0)/383;c3 = ([120 150 230]+128)/383;patch([0 1 1 0],[0 0 1 1],c1);patch([0 1 1 1-e 1-e 0+e],[0 0 1 1-e 0+e 0+e],c2);patch([0 0 1 1-e 0+e 0+e],[0 1 1 1-e 1-e 0+e],c3);plot([0 1 1 0 0],[0 0 1 1 0]);disp('Weights');
  "IW{1,1}(6,:)'" : Constant  Value=[0.483151554234079350091946025713696144521236419677734375;-0.49754981163547717937234438068117015063762664794921875;0.7441688497482179531772317204740829765796661376953125;-0.453430497902152229716676856696722097694873809814453125]
      mask Display: e = 0.06;c1 = [120 150 230]/255;c2 = ([120 150 230]+0)/383;c3 = ([120 150 230]+128)/383;patch([0 1 1 0],[0 0 1 1],c1);patch([0 1 1 1-e 1-e 0+e],[0 0 1 1-e 0+e 0+e],c2);patch([0 0 1 1-e 0+e 0+e],[0 1 1 1-e 1-e 0+e],c3);plot([0 1 1 0 0],[0 0 1 1 0]);disp('Weights');
  "IW{1,1}(7,:)'" : Constant  Value=[-0.8731909986143635560296161202131770551204681396484375;-0.065863625942295112025703929248265922069549560546875;0.0799641980758583059696320560760796070098876953125;-0.582106652013729242156614418490789830684661865234375]
      mask Display: e = 0.06;c1 = [120 150 230]/255;c2 = ([120 150 230]+0)/383;c3 = ([120 150 230]+128)/383;patch([0 1 1 0],[0 0 1 1],c1);patch([0 1 1 1-e 1-e 0+e],[0 0 1 1-e 0+e 0+e],c2);patch([0 0 1 1-e 0+e 0+e],[0 1 1 1-e 1-e 0+e],c3);plot([0 1 1 0 0],[0 0 1 1 0]);disp('Weights');
  "IW{1,1}(8,:)'" : Constant  Value=[0.6256753565606327782688822480849921703338623046875;0.1857796869207068157781037598397233523428440093994140625;0.317950172906602823719168782190536148846149444580078125;0.71373025450295968230562948519946075975894927978515625]
      mask Display: e = 0.06;c1 = [120 150 230]/255;c2 = ([120 150 230]+0)/383;c3 = ([120 150 230]+128)/383;patch([0 1 1 0],[0 0 1 1],c1);patch([0 1 1 1-e 1-e 0+e],[0 0 1 1-e 0+e 0+e],c2);patch([0 0 1 1-e 0+e 0+e],[0 1 1 1-e 1-e 0+e],c3);plot([0 1 1 0 0],[0 0 1 1 0]);disp('Weights');
  "IW{1,1}(9,:)'" : Constant  Value=[0.93884461394434548520138150706770829856395721435546875;-12.8543916671658582373538592946715652942657470703125;1.956732773586676632504577355575747787952423095703125;0.80749626182163158905069622051087208092212677001953125]
      mask Display: e = 0.06;c1 = [120 150 230]/255;c2 = ([120 150 230]+0)/383;c3 = ([120 150 230]+128)/383;patch([0 1 1 0],[0 0 1 1],c1);patch([0 1 1 1-e 1-e 0+e],[0 0 1 1-e 0+e 0+e],c2);patch([0 0 1 1-e 0+e 0+e],[0 1 1 1-e 1-e 0+e],c3);plot([0 1 1 0 0],[0 0 1 1 0]);disp('Weights');
  Mux : Mux  Inputs=15
      mask Display: e = 0.06;c1 = [120 150 230]/255;c2 = ([120 150 230]+0)/383;c3 = ([120 150 230]+128)/383;patch([0 1 1 0],[0 0 1 1],c1);patch([0 1 1 1-e 1-e 0+e],[0 0 1 1-e 0+e 0+e],c2);patch([0 0 1 1-e 0+e 0+e],[0 1 1 1-e 1-e 0+e],c3);plot([0 1 1 0 0],[0 0 1 1 0]);disp('Mux');
  dotprod{1..15} (15 alike) : neural/Weight Functions/dotprod
  "iz{1,1}" : Outport
      mask Display: e = 0.06;c1 = [120 230 180]/255;c2 = ([120 230 180]+0)/(256+128);c3 = ([120 230 180]+128)/(256+128);patch([0 1 1 0],[0 0 1 1],c1);patch([0 1 1 1-e 1-e 0+e],[0 0 1 1-e 0+e 0+e],c2);patch([0 0 1 1-e 0+e 0+e],[0 1 1 1-e 1-e 0+e],c3);plot([0 1 1 0 0],[0 0 1 1 0]);
  wires:
  Mux/1 -> "iz{1,1}"/1
  dotprod15/1 -> Mux/15
  "IW{1,1}(15,:)'"/1 -> dotprod15/1
  dotprod14/1 -> Mux/14
  "IW{1,1}(14,:)'"/1 -> dotprod14/1
  dotprod13/1 -> Mux/13
  "IW{1,1}(13,:)'"/1 -> dotprod13/1
  dotprod12/1 -> Mux/12
  "IW{1,1}(12,:)'"/1 -> dotprod12/1
  dotprod11/1 -> Mux/11
  "IW{1,1}(11,:)'"/1 -> dotprod11/1
  dotprod10/1 -> Mux/10
  "IW{1,1}(10,:)'"/1 -> dotprod10/1
  dotprod9/1 -> Mux/9
  "IW{1,1}(9,:)'"/1 -> dotprod9/1
  dotprod8/1 -> Mux/8
  "IW{1,1}(8,:)'"/1 -> dotprod8/1
  dotprod7/1 -> Mux/7
  "IW{1,1}(7,:)'"/1 -> dotprod7/1
  dotprod6/1 -> Mux/6
  "IW{1,1}(6,:)'"/1 -> dotprod6/1
  dotprod5/1 -> Mux/5
  "IW{1,1}(5,:)'"/1 -> dotprod5/1
  dotprod4/1 -> Mux/4
  "IW{1,1}(4,:)'"/1 -> dotprod4/1
  dotprod3/1 -> Mux/3
  "IW{1,1}(3,:)'"/1 -> dotprod3/1
  dotprod2/1 -> Mux/2
  "IW{1,1}(2,:)'"/1 -> dotprod2/1
  dotprod1/1 -> Mux/1
  "pd{1,1}"/1 -> dotprod15/2, dotprod14/2, dotprod13/2, dotprod12/2, dotprod11/2, dotprod10/2, dotprod9/2, dotprod8/2, dotprod7/2, dotprod6/2, dotprod5/2, dotprod4/2, dotprod3/2, dotprod2/2, dotprod1/2
  "IW{1,1}(1,:)'"/1 -> dotprod1/1
